simulink model "Model_Simu"  (R2023a)
settings: Solver=VariableStepAuto  StartTime=0.0  StopTime=10.0  RelTol=1e-3
values from neighbouring files (symbols this model uses):
  A = [ -(Re+R)/L,        -n1/(Ka*L*n2),   0,      0 ... (first row only)    [Model_PolePlacement.m]
  B = [ 1/L; 0; 0; 0 ]    [Model_PolePlacement.m]
  K = place(A,B,poles_desires)    [Model_PolePlacement.m]
  Kr = -1 / (C * inv(A - B*K) * B)    [Model_PolePlacement.m]
settings Model: Creator=Romai  LastModifiedBy=z92504359
settings RTWCC: GPUComputeCapability=5.0

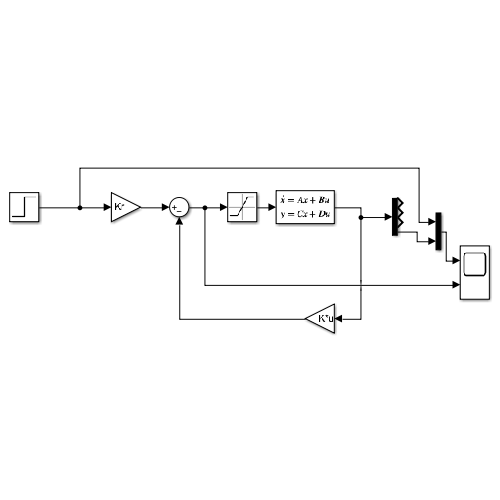
[thumbnail: Simulink's stored preview of the top-level diagram]
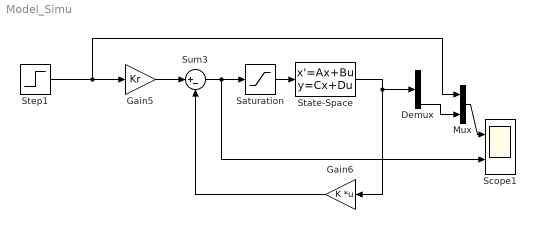
== system Model_Simu ==
  Demux : Demux
  Gain5 : Gain  Gain=Kr
  Gain6 : Gain  Gain=K  Multiplication=Matrix(K*u)
  Mux : Mux  Inputs=2
  Saturation : Saturate  UpperLimit=420  LowerLimit=-420
  Scope1 : Scope  NumInputPorts=2
  State-Space : StateSpace  A=A  B=B  C=eye(4)  D=zeros(4,1)  InitialCondition=0
  Step1 : Step  Time=0  After=10  SampleTime=0
  Sum3 : Sum  Inputs=|+-
  wires:
  State-Space/1 -> Demux/1, Gain6/1
  Gain5/1 -> Sum3/1
  Gain6/1 -> Sum3/2
  Step1/1 -> Mux/1, Gain5/1
  Sum3/1 -> Saturation/1, Scope1/2
  Demux/4 -> Mux/2
  Mux/1 -> Scope1/1
  Saturation/1 -> State-Space/1
